simulink model "vloop_test_4iii"  (R2025b)
settings: Solver=ode15s  StartTime=0.0  StopTime=3  RelTol=1e-3  EnableMultiTasking=on
InitFcn:
  | G = 107.815;
libraries: simulink x1, roblocks x1
Description:
  | vloop parameters for
  | Puma560 shoulder joint
  | with link inertia
  | RVC1 p.205
settings Model: DisableUpgradeWarningsForVersion=R2014b  Creator=pic  LastModifiedBy=ekkar
settings SolverCC: AlgebraicLoopSolver=TrustRegion
settings DataIOCC: LimitDataPoints=on  SaveFormat=Array  SignalLoggingSaveFormat=ModelDataLogs  TimeSaveName=t  OutputSaveName=y
settings OptimizationCC: ExpressionDepthLimit=2147483647.0  LifeSpan=inf
settings DebuggingCC: UnderspecifiedInitializationDetection=Classic  MergeDetectMultiDrivingBlocksExec=none  SolverPrmCheckMsg=warning  MultiTaskRateTransMsg=warning  FcnCallInpInsideContextMsg=warning  UnconnectedInputMsg=warning  UnconnectedOutputMsg=warning  UnconnectedLineMsg=warning  AllowSymbolicDim=off  StateNameClashWarn=warning  SFUnexpectedBacktrackingDiag=warning  SFNoUnconditionalDefaultTransitionDiag=warning  SFExecutionAtInitializationDiag=none  ArithmeticOperatorsInVariantConditions=warning
settings HardwareCC: ProdBitPerPointer=32.0  ProdBitPerSizeT=32.0  ProdBitPerPtrDiffT=32.0  ProdLargestAtomicFloat=None  ProdIntDivRoundTo=Undefined  ProdEndianess=Unspecified  ProdWordSize=32.0  ProdHWDeviceType=32-bit Generic
settings ModelReferenceCC: EnableRefExpFcnMdlSchedulingChecks=on  PropagateSignalLabelsOutOfModel=off
settings SFSimCC: SimUseLocalCustomCode=off  CustomCodeUndefinedFunction=UseInterfaceOnly
settings SFSimCC: SimCustomInitializer=|
  | if ~exist(tau_d)
  |    tau_d = 0
  | end
settings RTWCC: RTWUseLocalCustomCode=off  GPUComputeCapability=3.5
settings CodeAppCC: StateflowObjectComments=on
settings GRTTargetCC: TargetLangStandard=C89/C90 (ANSI)  CombineOutputUpdateFcns=off  GRTInterface=on
settings ConfigComp: CovMetricSettings=dw  CovSaveCumulativeToWorkspaceVar=on  CovSaveSingleToWorkspaceVar=on  CovExternalEMLEnable=off  CovSFcnEnable=off

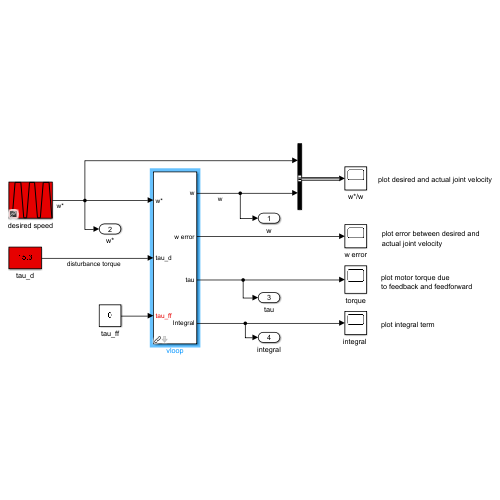
[thumbnail: Simulink's stored preview of the top-level diagram]
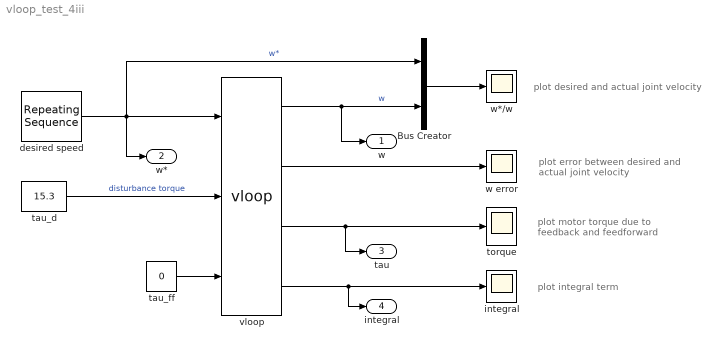
== system vloop_test_4iii ==
  note: plot integral term
  note: plot motor torque due
      | to feedback and feedforward
  note: plot error between desired and
      | actual joint velocity
  note: plot desired and actual joint velocity
  Bus Creator : BusCreator  Inputs=2
  desired speed : simulink/Sources/Repeating Sequence  rep_seq_t=[0 0.5 1 2 2.5]  rep_seq_y=[0 0 1 1 0]
  "integral " : Scope
      settings: TimeSpan=1  ActiveDisplayYMinimum=-88.121776999480559  ActiveDisplayYMaximum=50.509860613484726  DataLoggingVariableName=ScopeData3
  tau_d : Constant  Value=15.3
  tau_ff : Constant  Value=0
  torque : Scope
      settings: ActiveDisplayYMinimum=-127.76504352980145  ActiveDisplayYMaximum=188.79410164117758
  vloop : roblocks/Arm/vloop  J=39.3671  B=11.96  Km=1  tau_max=1e4  Kv=1562.7  Ki=0  T=0.001
  w error : Scope
      settings: ActiveDisplayString=4  ActiveDisplayYMinimum=-0.030915343900761911  ActiveDisplayYMaximum=0.013016518289212027  YLabel=torque  DataLoggingVariableName=ScopeData2
  w*/w : Scope
      settings: ActiveDisplayYMinimum=-0.13593093111603008  ActiveDisplayYMaximum=1.1262145479017811  YLabel=omega
  w : Outport
  w* : Outport  Port=2
  tau : Outport  Port=3
  integral : Outport  Port=4
  wires:
  Bus Creator/1 -> w*/w/1
  vloop/1 -> Bus Creator/2, w/1  "w"
  vloop/2 -> w error/1
  vloop/3 -> tau/1, torque/1
  vloop/4 -> integral/1, "integral "/1
  tau_d/1 -> vloop/2  "disturbance torque"
  tau_ff/1 -> vloop/3
  desired speed/1 -> Bus Creator/1, w*/1, vloop/1  "w*"
